simulink model "autotune_NFC2"  (R2026a)
settings: Solver=ode15s  StopTime=.004
StartFcn:
  | tic;
StopFcn:
  | trun_ss = toc
libraries: fl_lib x20, nesl_utility x6, ee_lib x2, simulink_extras x1, simulink x1
settings Model: SimulationMode=accelerator  Creator=kschutz  LastModifiedBy=kschutz
settings DataIOCC: InspectSignalLogs=on
settings OptimizationCC: SimCompilerOptimization=on
settings SimscapeCC: SimscapeNominalValues="[{\"value\":\"1\",\"unit\":\"A\"},{\"value\":\"1\",\"unit\":\"bar\"},{\"value\":\"1\",\"unit\":\"cm^2\"},{\"value\":\"1\",\"unit\":\"cm^3/s\"},{\"value\":\"1\",\"unit\":\"kJ/kg\"},{\"value\":\"1\",\"unit\":\"kW\"},{\"value\":\"1\",\"unit\":\"l\"},{\"value\":\"1\",\"unit\":\"N\"},{\"value\":\"1\",\"unit\":\"N*m\"},{\"value\":\"1\",\"unit\":\"V\"}]"  SimscapeLogType=none  SimscapeLogDataHistory=5000.0

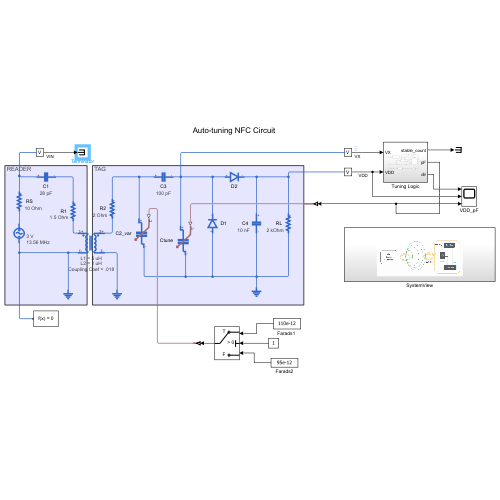
[thumbnail: Simulink's stored preview of the top-level diagram]
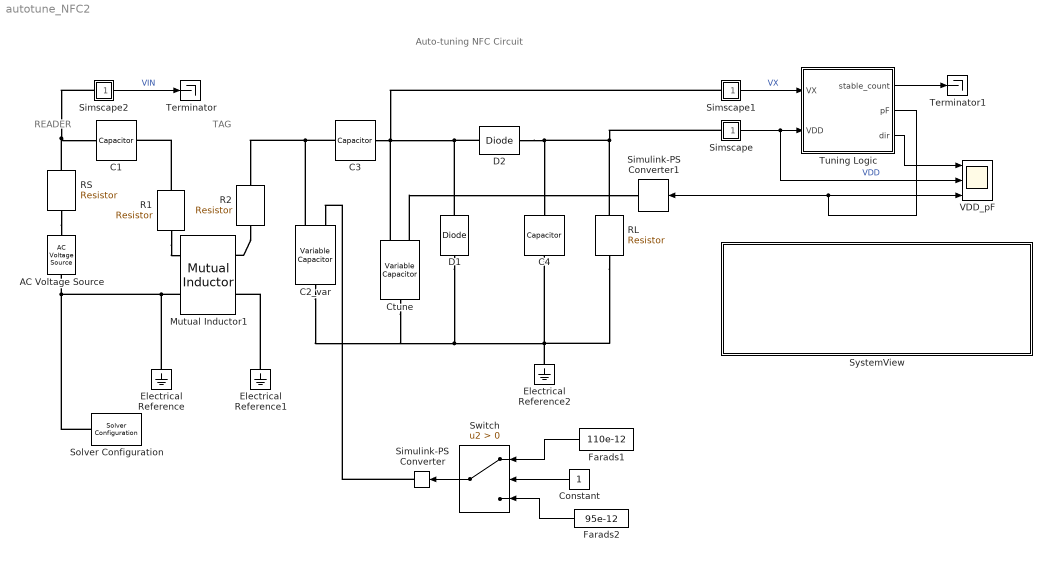
== system autotune_NFC2 ==
  note: TAG
  note: READER
  note: Auto-tuning NFC Circuit
  AC Voltage Source : fl_lib/Electrical/Electrical Sources/AC Voltage Source  amp=3 V  shift=0 deg  frequency=13.56 MHz
      settings: AttributesFormatString=|
      | %<amp> %<amp_unit>
      | %<frequency> %<frequency_unit>
  C1 : fl_lib/Electrical/Electrical Elements/Capacitor  c=28 pF  r=.1 Ohm  g=0 1/Ohm  i_specify=off  i_priority=None  i=0 A  i_nominal_specify=off  i_nominal_value=1  i_nominal_unit=A  v_specify=off  v_priority=None  v=0 V  v_nominal_specify=off  v_nominal_value=1  v_nominal_unit=V  vc_specify=off  vc_priority=High  vc=0 V  vc_nominal_specify=off  vc_nominal_value=1  vc_nominal_unit=V
      settings: AttributesFormatString=%<c> %<c_unit>
  C2_var : ee_lib/Passive/Variable Capacitor  prm=2  Cmin=.1 pF  r=.1 Ohm  v0=0 V  q0=0 C
  C3 : fl_lib/Electrical/Electrical Elements/Capacitor  c=100 pF  r=.1 Ohm  g=0 1/Ohm  i_specify=off  i_priority=None  i=0 A  i_nominal_specify=off  i_nominal_value=1  i_nominal_unit=A  v_specify=off  v_priority=None  v=0 V  v_nominal_specify=off  v_nominal_value=1  v_nominal_unit=V  vc_specify=off  vc_priority=High  vc=0 V  vc_nominal_specify=off  vc_nominal_value=1  vc_nominal_unit=V
      settings: AttributesFormatString=%<c> %<c_unit>
  C4 : fl_lib/Electrical/Electrical Elements/Capacitor  c=10 nF  r=1e-6 Ohm  g=0 1/Ohm  i_specify=off  i_priority=None  i=0 A  i_nominal_specify=off  i_nominal_value=1  i_nominal_unit=A  v_specify=off  v_priority=None  v=0 V  v_nominal_specify=off  v_nominal_value=1  v_nominal_unit=V  vc_specify=off  vc_priority=High  vc=0 V  vc_nominal_specify=off  vc_nominal_value=1  vc_nominal_unit=V
      settings: AttributesFormatString=%<c> %<c_unit>
  Constant : Constant
  Ctune : ee_lib/Passive/Variable Capacitor  prm=2  Cmin=.1 pF  r=.1 Ohm  v0=0 V  q0=0 C
  D1 : fl_lib/Electrical/Electrical Elements/Diode  Vf=0.6 V  Ron=0.3 Ohm  Goff=1e-8 1/Ohm  i_specify=off  i_priority=None  i=0 A  i_nominal_specify=off  i_nominal_value=1  i_nominal_unit=A  v_specify=off  v_priority=None  v=0 V  v_nominal_specify=off  v_nominal_value=1  v_nominal_unit=V
  D2 : fl_lib/Electrical/Electrical Elements/Diode  Vf=0.6 V  Ron=0.3 Ohm  Goff=1e-8 1/Ohm  i_specify=off  i_priority=None  i=0 A  i_nominal_specify=off  i_nominal_value=1  i_nominal_unit=A  v_specify=off  v_priority=None  v=0 V  v_nominal_specify=off  v_nominal_value=1  v_nominal_unit=V
  Electrical Reference : fl_lib/Electrical/Electrical Elements/Electrical Reference
  Electrical Reference1 : fl_lib/Electrical/Electrical Elements/Electrical Reference
  Electrical Reference2 : fl_lib/Electrical/Electrical Elements/Electrical Reference
  "Farads1 " : Constant  Value=110e-12
  Farads2 : Constant  Value=95e-12
  Mutual Inductor1 : fl_lib/Electrical/Electrical Elements/Mutual Inductor  L1=5 uH  L2=1 uH  perfectCoupling=false  k=.018  i1_specify=off  i1_priority=High  i1=0 A  i1_nominal_specify=off  i1_nominal_value=1  i1_nominal_unit=A  i2_specify=off  i2_priority=High  i2=0 A  i2_nominal_specify=off  i2_nominal_value=1  i2_nominal_unit=A  v1_specify=off  v1_priority=None  v1=0 V  v1_nominal_specify=off  v1_nominal_value=1  v1_nominal_unit=V  v2_specify=off  v2_priority=None  v2=0 V  v2_nominal_specify=off  v2_nominal_value=1  v2_nominal_unit=V
      settings: AttributesFormatString=|
      | L1 = %<L1> %<L1_unit>
      | L2 = %<L2> %<L2_unit>
      | Coupling Coef = %<k>
  R1 : fl_lib/Electrical/Electrical Elements/Resistor  R=1.5 Ohm  i_specify=off  i_priority=None  i=0 A  i_nominal_specify=off  i_nominal_value=1  i_nominal_unit=A  v_specify=off  v_priority=None  v=0 V  v_nominal_specify=off  v_nominal_value=1  v_nominal_unit=V
      settings: AttributesFormatString=%<R> %<R_unit>
  R2 : fl_lib/Electrical/Electrical Elements/Resistor  R=2 Ohm  i_specify=off  i_priority=None  i=0 A  i_nominal_specify=off  i_nominal_value=1  i_nominal_unit=A  v_specify=off  v_priority=None  v=0 V  v_nominal_specify=off  v_nominal_value=1  v_nominal_unit=V
      settings: AttributesFormatString=%<R> %<R_unit>
  RL : fl_lib/Electrical/Electrical Elements/Resistor  R=2 kOhm  i_specify=off  i_priority=None  i=0 A  i_nominal_specify=off  i_nominal_value=1  i_nominal_unit=A  v_specify=off  v_priority=None  v=0 V  v_nominal_specify=off  v_nominal_value=1  v_nominal_unit=V
      settings: AttributesFormatString=%<R> %<R_unit>
  RS : fl_lib/Electrical/Electrical Elements/Resistor  R=10 Ohm  i_specify=off  i_priority=None  i=0 A  i_nominal_specify=off  i_nominal_value=1  i_nominal_unit=A  v_specify=off  v_priority=None  v=0 V  v_nominal_specify=off  v_nominal_value=1  v_nominal_unit=V
      settings: AttributesFormatString=%<R> %<R_unit>
  Simscape : Subsystem
      mask Display: disp('V')
  Simscape1 : Subsystem
      mask Display: disp('V')
  Simscape2 : Subsystem
      mask Display: disp('V')
  Simulink-PS Converter : nesl_utility/Simulink-PS Converter  PhysicalDomain=network_engine_domain  SubClassName=ps_input  LeftPortType=input  RightPortType=output  PseudoPeriodic=off  Frequencies=[]  NoiseDistribution=none  NoiseParameters=[]  Unit=1  AffineConversion=off  FilteringAndDerivatives=provide  SimscapeFilterOrder=1  InputFilterTimeConstant=0.001  UdotUserProvided=0
  Simulink-PS Converter1 : nesl_utility/Simulink-PS Converter  PhysicalDomain=network_engine_domain  SubClassName=ps_input  LeftPortType=input  RightPortType=output  PseudoPeriodic=off  Frequencies=[]  NoiseDistribution=none  NoiseParameters=[]  Unit=1  AffineConversion=off  FilteringAndDerivatives=zero  SimscapeFilterOrder=1  InputFilterTimeConstant=.001  UdotUserProvided=0
  Solver Configuration : nesl_utility/Solver Configuration  PhysicalDomain=network_engine_domain  SubClassName=solver  LeftPortType=input  RightPortType=generic  Tones=[]  Harmonics=[]  SimulateNoise=off  Profile=off  UseLocalSampling=off  EnableSwitchedLinearOptims=on  FrequencyDomain=off  UseCCode=off  RelTol=0.001  AbsTol=1e-06  MinStep=1e-09  ToWorkspace=off  RevertToSquareIcSolve=off  NumHomotopyIterations=100  PhasorMode=off  PhasorModeNumHarmonics=1  ConsistencySolver=NEWTON_FTOL  CanonicalOrdering=UNORDERED  OptimizeIntermediates=UNOPTIMIZED  IndexReductionMethod=DerivativeReplacement  DoDC=off  ResidualTolerance=1e-09  ConsistencyTolSource=GLOBAL  ConsistencyAbsTol=0.001  ConsistencyRelTol=0.001  ConsistencyTolFactor=0.001  UseLocalSolver=on  LocalSolverChoice=NE_TRAPEZOIDAL_ADVANCER  ResolveIndetEquations=on  FunctionEvalNumThread=1  LocalSolverSampleTime=.01/13.56e6  DoFixedCost=off  MaxNonlinIter=3  MaxModeIter=2  ComputeImpulses=off  ImpulseIterations=2  LinearAlgebra=Sparse  LinearAlgebraNumThread=0  EquationFormulation=NE_TIME_EF  DelaysMemoryBudget=1024  AutomaticFiltering=on  FilteringTimeConstant=0.001  PartitionStorageMethod=AS_NEEDED  PartitionMemoryBudget=1024  PartitionMethod=FAST  MultibodyUseLocalSolver=off  MultibodyLocalSolverChoice=ODE1  MultibodyLocalSolverSampleTime=0.001
  Switch : Switch  Criteria=u2 > Threshold  SaturateOnIntegerOverflow=off  InputSameDT=off
  SystemView : Subsystem
  Terminator : Terminator
  Terminator1 : Terminator
  Tuning Logic : Subsystem
  VDD_pF : Scope  NumInputPorts=3
      settings: ActiveDisplayYMinimum=-1.25  ActiveDisplayYMaximum=1.25
  wires:
  Simscape2/1(Out) -> Terminator/1  "VIN"
  Switch/1 -> Simulink-PS Converter/1
  Constant/1 -> Switch/2
  "Farads1 "/1 -> Switch/1
  Farads2/1 -> Switch/3
  Simscape1/1(Out) -> Tuning Logic/1(VX)  "VX"
  Simscape/1(Out) -> VDD_pF/2, Tuning Logic/2(VDD)  "VDD"
  Tuning Logic/1(stable_count) -> Terminator1/1
  Tuning Logic/2(pF) -> Simulink-PS Converter1/1, VDD_pF/3
  Tuning Logic/3(dir) -> VDD_pF/1
  connections:
  Electrical Reference/LConn1 -- Mutual Inductor1/LConn2 -- Solver Configuration/RConn1 -- AC Voltage Source/RConn1
  R1/LConn1 -- C1/RConn1
  R1/RConn1 -- Mutual Inductor1/LConn1
  R2/RConn1 -- Mutual Inductor1/RConn1
  C2_var/RConn1 -- Ctune/RConn1 -- D1/LConn1 -- RL/RConn1 -- Electrical Reference2/LConn1 -- C4/RConn1
  Simscape/LConn1 -- RL/LConn1 -- D2/RConn1 -- C4/LConn1
  Electrical Reference1/LConn1 -- Mutual Inductor1/RConn2
  C3/LConn1 -- R2/LConn1 -- C2_var/LConn2
  Ctune/LConn1 -- Simulink-PS Converter1/RConn1
  Simscape2/LConn1 -- C1/LConn1 -- RS/LConn1
  Ctune/LConn2 -- Simscape1/LConn1 -- D2/LConn1 -- D1/RConn1 -- C3/RConn1
  RS/RConn1 -- AC Voltage Source/LConn1
  Simulink-PS Converter/RConn1 -- C2_var/LConn1

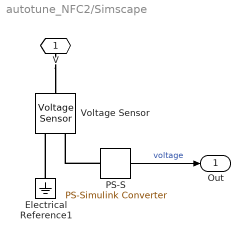
== system autotune_NFC2/Simscape ==
  Electrical Reference1 : fl_lib/Electrical/Electrical Elements/Electrical Reference
  PS-S : nesl_utility/PS-Simulink Converter  PhysicalDomain=network_engine_domain  SubClassName=ps_output  LeftPortType=input  RightPortType=output  PseudoPeriodic=off  Frequencies=[]  VectorFormat=1-D array  Unit=V  AffineConversion=off
  Voltage Sensor : fl_lib/Electrical/Electrical Sensors/Voltage Sensor
  V : PMIOPort  Side=Left
  Out : Outport  VectorParamsAs1DForOutWhenUnconnected=off
  wires:
  PS-S/1 -> Out/1  "voltage"
  connections:
  PS-S/LConn1 -- Voltage Sensor/RConn1
  V/RConn1 -- Voltage Sensor/LConn1
  Electrical Reference1/LConn1 -- Voltage Sensor/RConn2

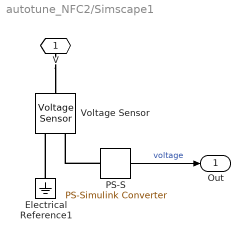
== system autotune_NFC2/Simscape1 ==
  Electrical Reference1 : fl_lib/Electrical/Electrical Elements/Electrical Reference
  PS-S : nesl_utility/PS-Simulink Converter  PhysicalDomain=network_engine_domain  SubClassName=ps_output  LeftPortType=input  RightPortType=output  PseudoPeriodic=off  Frequencies=[]  VectorFormat=1-D array  Unit=V  AffineConversion=off
  Voltage Sensor : fl_lib/Electrical/Electrical Sensors/Voltage Sensor
  V : PMIOPort  Side=Left
  Out : Outport  VectorParamsAs1DForOutWhenUnconnected=off
  wires:
  PS-S/1 -> Out/1  "voltage"
  connections:
  PS-S/LConn1 -- Voltage Sensor/RConn1
  V/RConn1 -- Voltage Sensor/LConn1
  Electrical Reference1/LConn1 -- Voltage Sensor/RConn2

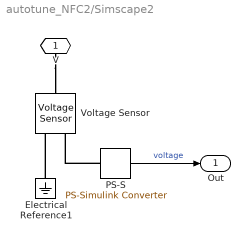
== system autotune_NFC2/Simscape2 ==
  Electrical Reference1 : fl_lib/Electrical/Electrical Elements/Electrical Reference
  PS-S : nesl_utility/PS-Simulink Converter  PhysicalDomain=network_engine_domain  SubClassName=ps_output  LeftPortType=input  RightPortType=output  PseudoPeriodic=off  Frequencies=[]  VectorFormat=1-D array  Unit=V  AffineConversion=off
  Voltage Sensor : fl_lib/Electrical/Electrical Sensors/Voltage Sensor
  V : PMIOPort  Side=Left
  Out : Outport  VectorParamsAs1DForOutWhenUnconnected=off
  wires:
  PS-S/1 -> Out/1  "voltage"
  connections:
  Electrical Reference1/LConn1 -- Voltage Sensor/RConn2
  V/RConn1 -- Voltage Sensor/LConn1
  PS-S/LConn1 -- Voltage Sensor/RConn1

== system autotune_NFC2/SystemView ==

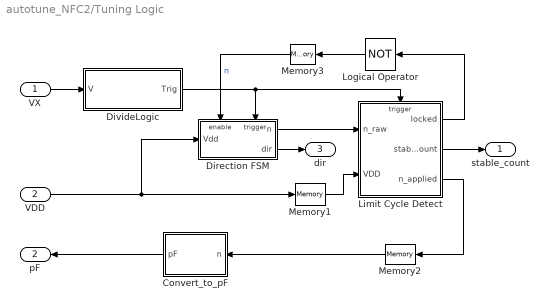
== system autotune_NFC2/Tuning Logic ==
  VX : Inport
  VDD : Inport  Port=2
  Convert_to_pF : Subsystem
  Direction FSM : Subsystem
  DivideLogic : Subsystem
  Limit Cycle Detect : Stateflow chart  TreatAsAtomicUnit=on
  Logical Operator : Logic  Operator=NOT  AllPortsSameDT=off  OutDataTypeStr=boolean
  "Memory1 " : Memory
  "Memory2 " : Memory
  "Memory3 " : Memory
  stable_count : Outport
  pF : Outport  Port=2
  dir : Outport  Port=3
  wires:
  VDD/1 -> Direction FSM/1(Vdd), "Memory1 "/1
  DivideLogic/1(Trig) -> Direction FSM/Trigger, Limit Cycle Detect/Trigger
  "Memory1 "/1 -> Limit Cycle Detect/2(VDD)
  Logical Operator/1 -> "Memory3 "/1
  VX/1 -> DivideLogic/1(V)
  Limit Cycle Detect/1(locked) -> Logical Operator/1
  "Memory3 "/1 -> Direction FSM/Enable  "n"
  Limit Cycle Detect/3(n_applied) -> "Memory2 "/1
  Limit Cycle Detect/2(stable_count) -> stable_count/1
  "Memory2 "/1 -> Convert_to_pF/1(n)
  Direction FSM/1(n) -> Limit Cycle Detect/1(n_raw)
  Convert_to_pF/1(pF) -> pF/1
  Direction FSM/2(dir) -> dir/1

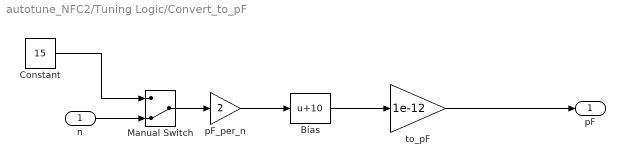
== system autotune_NFC2/Tuning Logic/Convert_to_pF ==
  n : Inport
  Bias : Bias  Bias=10  SaturateOnIntegerOverflow=off
  Constant : Constant  Value=15
  Manual Switch : ManualSwitch  CurrentSetting=0
  pF_per_n : Gain  Gain=2
  to_pF : Gain  Gain=1e-12
  pF : Outport  VectorParamsAs1DForOutWhenUnconnected=off
  wires:
  pF_per_n/1 -> Bias/1
  Bias/1 -> to_pF/1
  n/1 -> Manual Switch/2
  Manual Switch/1 -> pF_per_n/1
  Constant/1 -> Manual Switch/1
  to_pF/1 -> pF/1

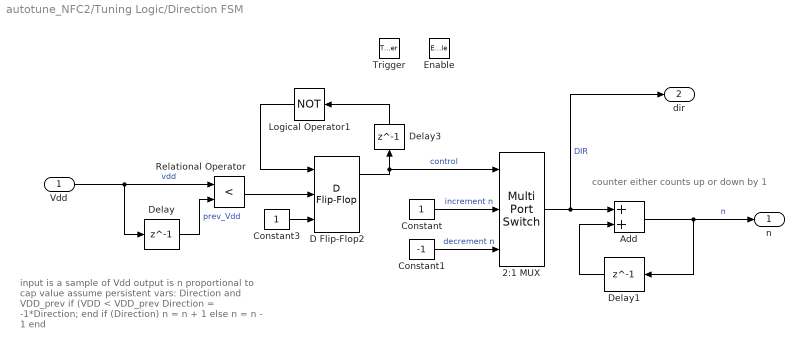
== system autotune_NFC2/Tuning Logic/Direction FSM ==
  note: input is a sample of Vdd
      | output is n proportional to cap value
      | assume persistent vars: Direction and VDD_prev
      |
      | if (VDD < VDD_prev
      |   Direction = -1*Direction;
      | end
      | if (Direction)
      | 	n = n + 1
      | else
      | 	n = n - 1
      | end
  note: counter either counts up or down by 1
  Vdd : Inport
  Enable : EnablePort
  Trigger : TriggerPort  VariantControl=Variant  PortDimensions=1
  2:1 MUX : MultiPortSwitch  DataPortOrder=Zero-based contiguous  Inputs=2  zeroidx=on  SaturateOnIntegerOverflow=off  InputSameDT=off
  Add : Sum
  Constant : Constant
  Constant1 : Constant  Value=-1
  Constant3 : Constant
  D Flip-Flop2 : simulink_extras/Flip Flops/D Flip-Flop
  Delay : Delay  DelayLength=1
  Delay1 : Delay  DelayLength=1  InitialCondition=17
      settings: AttributesFormatString=init = %<InitialCondition>
  Delay3 : Delay  DelayLength=1  InitialCondition=0
  Logical Operator1 : Logic  Operator=NOT  AllPortsSameDT=off  OutDataTypeStr=boolean
  Relational Operator : RelationalOperator  Operator=<  OutDataTypeStr=boolean  RndMeth=Simplest  InputSameDT=off
  n : Outport  VectorParamsAs1DForOutWhenUnconnected=off
  dir : Outport  Port=2  VectorParamsAs1DForOutWhenUnconnected=off
  wires:
  Relational Operator/1 -> D Flip-Flop2/2
  Delay3/1 -> Logical Operator1/1
  Logical Operator1/1 -> D Flip-Flop2/1
  D Flip-Flop2/1 -> Delay3/1, 2:1 MUX/1  "control"
  Constant3/1 -> D Flip-Flop2/3
  Vdd/1 -> Relational Operator/1, Delay/1  "vdd"
  Constant/1 -> 2:1 MUX/2  "increment n"
  Constant1/1 -> 2:1 MUX/3  "decrement n"
  Delay/1 -> Relational Operator/2  "prev_Vdd"
  Delay1/1 -> Add/2
  Add/1 -> Delay1/1, n/1  "n"
  2:1 MUX/1 -> dir/1, Add/1  "DIR"

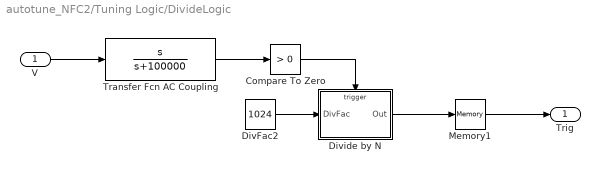
== system autotune_NFC2/Tuning Logic/DivideLogic ==
  V : Inport
  Compare To Zero : simulink/Logic and Bit Operations/Compare To Zero  relop=>  OutDataTypeStr=boolean
  DivFac2 : Constant  Value=1024
  Divide by N : Subsystem  TreatAsAtomicUnit=on
  Memory1 : Memory
  Transfer Fcn AC Coupling : TransferFcn  Numerator=[1 0]  Denominator=[1 100000]
  Trig : Outport  VectorParamsAs1DForOutWhenUnconnected=off
  wires:
  Memory1/1 -> Trig/1
  V/1 -> Transfer Fcn AC Coupling/1
  Compare To Zero/1 -> Divide by N/Trigger
  Divide by N/1(Out) -> Memory1/1
  Transfer Fcn AC Coupling/1 -> Compare To Zero/1
  DivFac2/1 -> Divide by N/1(DivFac)

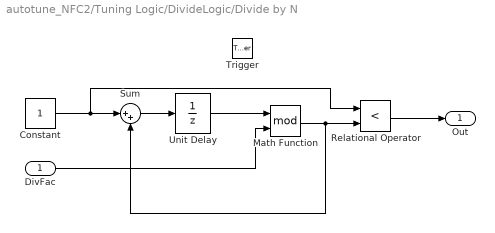
== system autotune_NFC2/Tuning Logic/DivideLogic/Divide by N ==
  DivFac : Inport
  Trigger : TriggerPort  VariantControl=Variant  PortDimensions=1
  Constant : Constant
  Math Function : Math  Operator=mod  SignedPower=on
  Relational Operator : RelationalOperator  Operator=<
  Sum : Sum  Inputs=|++  InputSameDT=on  SaturateOnIntegerOverflow=on  OutDataTypeStr=Inherit: Same as first input
  Unit Delay : UnitDelay  SampleTime=-1
  Out : Outport  VectorParamsAs1DForOutWhenUnconnected=off
  wires:
  Relational Operator/1 -> Out/1
  Math Function/1 -> Relational Operator/2, Sum/2
  DivFac/1 -> Math Function/2
  Unit Delay/1 -> Math Function/1
  Sum/1 -> Unit Delay/1
  Constant/1 -> Relational Operator/1, Sum/1

== stateflow chart autotune_NFC2/Tuning Logic/Limit Cycle Detect ==
  state Initialize
    en:
    locked = false;
    n_min = n_raw;
    n_max = n_raw;
    stable_count = 0;
    VDD_ref = VDD;
    n_applied = n_raw;
  state Seeking
    n_min = min(n_min, n_raw);
    n_max = max(n_max, n_raw);
    if n_max - n_min <= 3
    stable_count = stable_count + 1;
    else
    n_min = n_raw;
    n_max = n_raw;
    stable_count = 0;
    end
    n_applied = n_raw;
  state Locked
  (default) -> Initialize
  Initialize -> Seeking : [true]
  Seeking -> Locked : [stable_count >= 7] /{ locked = true; VDD_ref = VDD; n_applied = n_raw;}
  Locked -> Seeking : [VDD < 0.90 * VDD_ref || VDD > 1.10 * VDD_ref] /{ locked = false; n_min = n_raw; n_max = n_raw; stable_count = 0;}
  data: locked output boolean size=1 =false; n_raw input double size=1; VDD input double size=1; n_min local double size=1 =0; n_max local double size=1 =0; VDD_ref local double size=1 =0; stable_count output double size=1 =0; n_applied output double size=1 =0
  events: trigger_update input RISING_EDGE_EVENT
